simulink model "FOCwithLOAD"  (R2024b)
settings: Solver=FixedStepDiscrete  StartTime=0.0  StopTime=inf  RelTol=1e-3
PreLoadFcn:
  | % 自动加载同目录下的 linear_data.m，确保换机/首次打开可直接更新与编译
  | if ~evalin('base', 'exist(''Ts'',''var'') && exist(''pmsm'',''var'') && exist(''SMRC_I_Vsat_thresh'',''var'')')
  |     mdlDir_ = '';
  |     if bdIsLoaded('FOCwithLOAD'), mdlDir_ = fileparts(get_param('FOCwithLOAD', 'FileName')); end
  |     if isempty(mdlDir_), mdlDir_ = fileparts(which('FOCwithLOAD')); end
  |     if isempty(mdlDir_), mdlDir_ = pwd; end
  |     dataFile_ = fullfile(mdlDir_, 'linear_data.m');
  |     if isfile(dataFile_)
  |         assignin('base', 'linearDataFileTmp_', dataFile_);
  |         evalin('base', 'run(linearDataFileTmp_); clear linearDataFileTmp_');
  |     end
  |     clear mdlDir_ dataFile_
  | end
InitFcn:
  | % 自动加载同目录下的 linear_data.m，确保换机/首次打开可直接更新与编译
  | if ~evalin('base', 'exist(''Ts'',''var'') && exist(''pmsm'',''var'') && exist(''SMRC_I_Vsat_thresh'',''var'')')
  |     mdlDir_ = '';
  |     if bdIsLoaded('FOCwithLOAD'), mdlDir_ = fileparts(get_param('FOCwithLOAD', 'FileName')); end
  |     if isempty(mdlDir_), mdlDir_ = fileparts(which('FOCwithLOAD')); end
  |     if isempty(mdlDir_), mdlDir_ = pwd; end
  |     dataFile_ = fullfile(mdlDir_, 'linear_data.m');
  |     if isfile(dataFile_)
  |         assignin('base', 'linearDataFileTmp_', dataFile_);
  |         evalin('base', 'run(linearDataFileTmp_); clear linearDataFileTmp_');
  |     end
  |     clear mdlDir_ dataFile_
  | end
values from neighbouring files (symbols this model uses):
  a_hat = Kt_eff / (pmsm.J * omega_pu_base)    [linear_data.m]
  ADRC_B0 = 6055    [linear_data.m]
  ADRC_Wc = 3.2e-3    (= 0.0032)    [linear_data.m]
  ADRC_Wo = 30    [linear_data.m]
  alpha_ppc = exp(-lambda_ppc*Ts_speed)    [linear_data.m]
  b_hat = pmsm.B/pmsm.J    [linear_data.m]
  beta1 = single(2.0 * w_o)    [linear_data.m]
  beta2_sat_scale = 0.2    [linear_data.m]
  dataType = 'single'    [linear_data.m]
  gamma_reset = 0.9    [linear_data.m]
  inv_a_hat = 1/double(a_hat)    [linear_data.m]
  k_xi = 55    [linear_data.m]
  Kff = 0.98931745    [linear_data.m]
  lambda_ppc = 45    [linear_data.m]
  P_inf_const = 0.004    [linear_data.m]
  PI_params = mcb_SetControllerParameters(pmsm,inverter,PU_System,T_pwm,Ts,Ts_speed)    [linear_data.m]
  pmsm2 = pmsm    [linear_data.m]
  s_limit_sat = 0.9    [linear_data.m]
  speedRPM2mmps = pmlsm.mmps_per_rpm    [linear_data.m]
  target = mcb_SetProcessorDetails('F28379D',PWM_frequency)    [linear_data.m]
  Ts = T_pwm    (= 5e-05)    [linear_data.m]
  Ts_motor = T_pwm/2    (= 2.5e-05)    [linear_data.m]
  Ts_speed = 1*Ts    (= 5e-05)    [linear_data.m]
  w_o = single(200.0)    [linear_data.m]
  z2_limit = single(100.0)    [linear_data.m]
undefined symbols (not defined in the file or in its folder): DiscIntNeverNeededParam, Down, GPTRIP1SEL, GPTRIP2SEL, innerPI, inverter, inverter2, outerPI, pmlsm, pmsm, Tctr, TZ1, TZ2, Up
libraries: c2802xlib x13, simulink x10, c2837xDlib x6, c280xlib x6, slpidlib x5, svdschedulerlib x4, mcbcontrolslib x4, mcbpositiondecoderlib x2, mcbpmsmnonlinearlib x2, autolibpmsmexterior x2, mcbplantlib x2, svdutilitieslib x1
(part 1 of 5)
settings Model: ExtModeTrigDuration=8  Creator=The MathWorks, Inc.  LastModifiedBy=admin
settings SolverCC: AlgebraicLoopSolver=TrustRegion  MaxZcPerStep=1
settings OptimizationCC: DefaultParameterBehavior=Inlined  DefaultUnderspecifiedDataType=single  ReuseModelBlockBuffer=off  EnhancedBackFolding=on  InitFltsAndDblsToZero=on  NoFixptDivByZeroProtection=on  EfficientFloat2IntCast=on  EfficientMapNaN2IntZero=off  MaxStackSize=1024  OptimizeBlockOrder=speed  DifferentSizesBufferReuse=on  DenormalBehavior=FlushToZero  EfficientTunableParamExpr=on
settings DebuggingCC: MultiTaskDSMMsg=none  ParameterPrecisionLossMsg=none  ParameterTunabilityLossMsg=error  UnconnectedInputMsg=warning  UnconnectedOutputMsg=warning  UnconnectedLineMsg=warning
settings HardwareCC: ProdBitPerChar=16  ProdBitPerInt=16  ProdBitPerPointer=32  ProdBitPerSizeT=32  ProdBitPerPtrDiffT=32  ProdLargestAtomicInteger=Integer  ProdLargestAtomicFloat=None  ProdWordSize=16  ProdLongLongMode=on  ProdHWDeviceType=Texas Instruments->C2000
settings ModelReferenceCC: EnableRefExpFcnMdlSchedulingChecks=on
settings SFSimCC: MATLABDynamicMemAlloc=off
settings RTWCC: Description=Embedded Coder  SystemTargetFile=ert.tlc  HardwareBoard=TI Delfino F28379D LaunchPad  TemplateMakefile=ert_default_tmf  GenerateReport=on  Toolchain=Texas Instruments Code Composer Studio (C2000)  BuildConfiguration=Faster Runs  GPUComputeCapability=3.5  DLArmComputeVersion=19.05
settings CodeAppCC: IgnoreCustomStorageClasses=off  StateflowObjectComments=on
settings ERTTargetCC: CodeReplacementLibrary=TI C28x  ExtModeStaticAllocSize=10000  InlinedParameterPlacement=Hierarchical  ConvertIfToSwitch=off  SuppressUnreachableDefaultCases=off  MemSecPackage=tic2000demospkg  DynamicArrayContainerType=coder::array

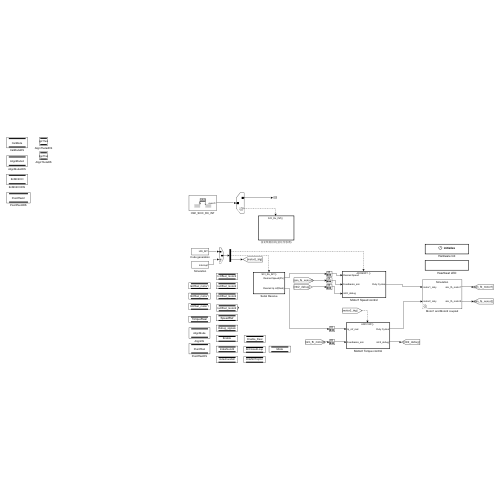
[thumbnail: Simulink's stored preview of the top-level diagram]
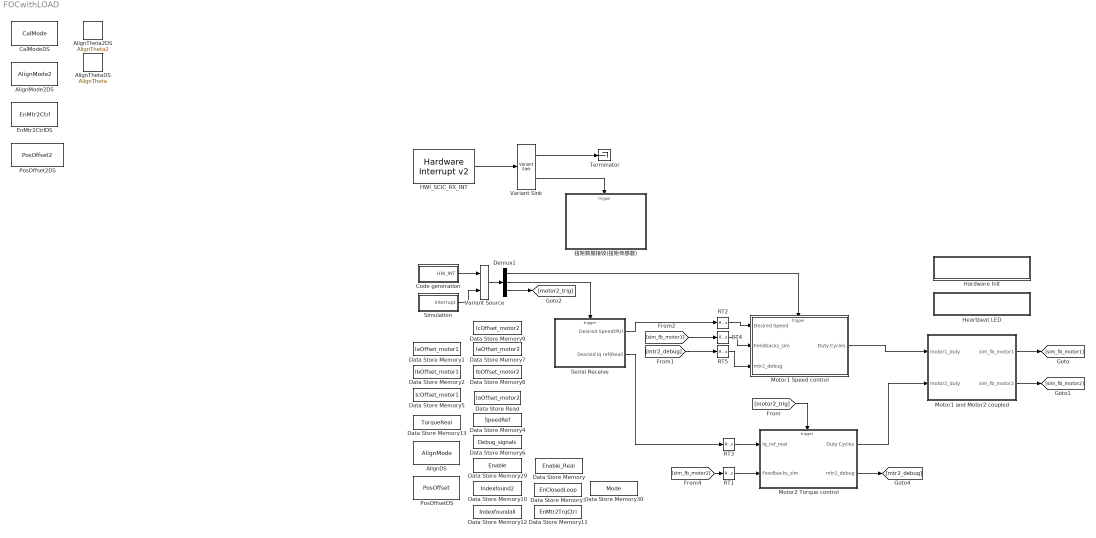
== system FOCwithLOAD ==
  AlignDS : DataStoreMemory  DataStoreName=AlignMode  WriteAfterWriteMsg=warning  ShowAdditionalParam=off  OutDataTypeStr=boolean
  AlignMode2DS : DataStoreMemory  DataStoreName=AlignMode2  WriteAfterWriteMsg=warning  ShowAdditionalParam=off  OutDataTypeStr=boolean
  AlignTheta2DS : DataStoreMemory  DataStoreName=AlignTheta2  WriteAfterWriteMsg=warning  ShowAdditionalParam=off  OutDataTypeStr=single
  AlignThetaDS : DataStoreMemory  DataStoreName=AlignTheta  WriteAfterWriteMsg=warning  ShowAdditionalParam=off  OutDataTypeStr=single
  CalModeDS : DataStoreMemory  DataStoreName=CalMode  WriteAfterWriteMsg=warning  ShowAdditionalParam=off  OutDataTypeStr=uint8
  Code generation : Subsystem
  Data Store Memory : DataStoreMemory  DataStoreName=Enable_Real  WriteAfterWriteMsg=warning  ShowAdditionalParam=off
  Data Store Memory1 : DataStoreMemory  DataStoreName=IaOffset_motor1  ReadBeforeWriteMsg=warning  WriteAfterWriteMsg=warning  WriteAfterReadMsg=warning  InitialValue=inverter.CtSensAOffset  ShowAdditionalParam=off
  Data Store Memory10 : DataStoreMemory  DataStoreName=Indexfound2  ReadBeforeWriteMsg=warning  WriteAfterWriteMsg=warning  WriteAfterReadMsg=warning  ShowAdditionalParam=off  OutDataTypeStr=boolean
  Data Store Memory11 : DataStoreMemory  DataStoreName=EnMtr2TrqCtrl  ReadBeforeWriteMsg=warning  WriteAfterWriteMsg=warning  WriteAfterReadMsg=warning  ShowAdditionalParam=off  OutDataTypeStr=boolean
  Data Store Memory12 : DataStoreMemory  DataStoreName=Indexfoundall  ReadBeforeWriteMsg=warning  WriteAfterWriteMsg=warning  WriteAfterReadMsg=warning  ShowAdditionalParam=off  OutDataTypeStr=boolean
  Data Store Memory13 : DataStoreMemory  DataStoreName=TorqueReal  InitialValue=1  ShowAdditionalParam=off  OutDataTypeStr=single
  Data Store Memory2 : DataStoreMemory  DataStoreName=IbOffset_motor1  ReadBeforeWriteMsg=warning  WriteAfterWriteMsg=warning  WriteAfterReadMsg=warning  InitialValue=inverter.CtSensBOffset  ShowAdditionalParam=off
  Data Store Memory29 : DataStoreMemory  DataStoreName=Enable  ReadBeforeWriteMsg=warning  WriteAfterWriteMsg=warning  WriteAfterReadMsg=warning  ShowAdditionalParam=off  OutDataTypeStr=boolean
  Data Store Memory3 : DataStoreMemory  DataStoreName=EnClosedLoop  ReadBeforeWriteMsg=warning  WriteAfterWriteMsg=warning  WriteAfterReadMsg=warning  ShowAdditionalParam=off  OutDataTypeStr=boolean
  Data Store Memory4 : DataStoreMemory  DataStoreName=SpeedRef  ShowAdditionalParam=off
  Data Store Memory5 : DataStoreMemory  DataStoreName=IcOffset_motor1  ReadBeforeWriteMsg=warning  WriteAfterWriteMsg=warning  WriteAfterReadMsg=warning  InitialValue=inverter.CtSensCOffset  ShowAdditionalParam=off
  Data Store Memory6 : DataStoreMemory  DataStoreName=Debug_signals  ReadBeforeWriteMsg=warning  WriteAfterWriteMsg=warning  WriteAfterReadMsg=warning  InitialValue=5  ShowAdditionalParam=off  OutDataTypeStr=uint16
  Data Store Memory7 : DataStoreMemory  DataStoreName=IaOffset_motor2  ReadBeforeWriteMsg=warning  WriteAfterWriteMsg=warning  WriteAfterReadMsg=warning  InitialValue=inverter2.CtSensAOffset  ShowAdditionalParam=off
  Data Store Memory8 : DataStoreMemory  DataStoreName=IbOffset_motor2  ReadBeforeWriteMsg=warning  WriteAfterWriteMsg=warning  WriteAfterReadMsg=warning  InitialValue=inverter2.CtSensBOffset  ShowAdditionalParam=off
  Data Store Memory9 : DataStoreMemory  DataStoreName=IcOffset_motor2  ReadBeforeWriteMsg=warning  WriteAfterWriteMsg=warning  WriteAfterReadMsg=warning  InitialValue=inverter2.CtSensCOffset  ShowAdditionalParam=off
  Data Store Read : DataStoreRead  DataStoreName=IaOffset_motor2  IndexOptions=Index vector (dialog)  Indices=1  OutputSizes=1
  Data Store Memory30 : DataStoreMemory  DataStoreName=Mode  ReadBeforeWriteMsg=warning  WriteAfterWriteMsg=warning  WriteAfterReadMsg=warning  InitialValue=uint16(0)  ShowAdditionalParam=off  OutDataTypeStr=uint16
  Demux1 : Demux  Outputs=3
  EnMtr2CtrlDS : DataStoreMemory  DataStoreName=EnMtr2Ctrl  WriteAfterWriteMsg=warning  ShowAdditionalParam=off  OutDataTypeStr=boolean
  HWI_SCIC_RX_INT : svdschedulerlib/Hardware Interrupt v2  ISRGroup=ADC - Analog to Digital Converter  ISRName=ADCA1_INT  ISRNumber=32  NumEventsToServe=1  EventsList={'on','EOC event','1';'off','Overflow event','2';'off','Custom event','3'}  SelectedEvents={'event1'}  TaskPriority=20  DisablePreemption=on  ClearInterruptFlagsAtEndOfEvent=on  InterruptDefinitionFile=$(TARGET_ROOT)/registry/interrupts/F2837xS_interrupts.xml  HardwareBoard=F2837x  EnableSimPort=off
      settings: LibrarySourceBlock=c2000lib/Scheduling/Hardware Interrupt
  Hardware Init : Subsystem  TreatAsAtomicUnit=on
  Heartbeat LED : Subsystem  TreatAsAtomicUnit=on
  Motor1 Speed control : Subsystem
      settings: RTWSystemCode=Nonreusable function
  Motor1 and Motor2 coupled : Subsystem  Variant=on  VariantControlMode=sim codegen switching  VariantControl=Motor1 and Motor2 coupled
  Motor2 Torque control : Subsystem
      settings: RTWSystemCode=Nonreusable function
  PosOffset2DS : DataStoreMemory  DataStoreName=PosOffset2  WriteAfterWriteMsg=warning  ShowAdditionalParam=off  OutDataTypeStr=single
  PosOffsetDS : DataStoreMemory  DataStoreName=PosOffset  WriteAfterWriteMsg=warning  ShowAdditionalParam=off  OutDataTypeStr=single
  RT{1..5} (5 alike) : RateTransition  Deterministic=off
  Serial Receive : Subsystem  SystemSampleTime=1e-3
  Simulation : Subsystem
  Terminator : Terminator
  Variant Sink : VariantSink  VariantControlMode=sim codegen switching
  Variant Source : VariantSource  VariantControlMode=sim codegen switching  OutputFunctionCall=on
  扭矩数据接收(扭矩传感器) : Subsystem  SystemSampleTime=1e-3
  wires:
  RT4/1 -> Motor1 Speed control/2(Feedbacks_sim)
  [sim_fb_motor1] -> RT4/1
  Simulation/1(Interrupt) -> Variant Source/2
  Code generation/1(HW_INT) -> Variant Source/1
  Variant Source/1 -> Demux1/1
  Demux1/1 -> Motor1 Speed control/Trigger
  Demux1/2 -> Serial Receive/Trigger
  Demux1/3 -> [motor2_trig]
  [motor2_trig] -> Motor2 Torque control/Trigger
  [sim_fb_motor2] -> RT1/1
  RT1/1 -> Motor2 Torque control/2(Feedbacks_sim)
  Serial Receive/1(Desired Speed(PU)) -> RT2/1
  Serial Receive/2(Desried Iq ref(Real)) -> RT3/1
  RT2/1 -> Motor1 Speed control/1(Desired Speed)
  RT3/1 -> Motor2 Torque control/1(Iq_ref_real)
  Motor2 Torque control/2(mtr2_debug) -> [mtr2_debug]
  [mtr2_debug] -> RT5/1
  RT5/1 -> Motor1 Speed control/3(mtr2_debug)
  HWI_SCIC_RX_INT/1 -> Variant Sink/1
  Variant Sink/2 -> 扭矩数据接收(扭矩传感器)/Trigger
  Variant Sink/1 -> Terminator/1
  Motor1 Speed control/1(Duty Cycles) -> Motor1 and Motor2 coupled/1(motor1_duty)
  Motor2 Torque control/1(Duty Cycles) -> Motor1 and Motor2 coupled/2(motor2_duty)
  Motor1 and Motor2 coupled/1(sim_fb_motor1) -> [sim_fb_motor1]
  Motor1 and Motor2 coupled/2(sim_fb_motor2) -> [sim_fb_motor2]

== system FOCwithLOAD/Code generation ==
  HWI_ADCB1_INT : svdschedulerlib/Hardware Interrupt v2  ISRGroup=ADC - Analog to Digital Converter  ISRName=ADCA1_INT  ISRNumber=32  NumEventsToServe=1  EventsList={'on','EOC event','1';'off','Overflow event','2';'off','Custom event','3'}  SelectedEvents={'event1'}  TaskPriority=30  DisablePreemption=off  ClearInterruptFlagsAtEndOfEvent=on  InterruptDefinitionFile=$(TARGET_ROOT)/registry/interrupts/F2837xS_interrupts.xml  HardwareBoard=F2837x  EnableSimPort=off
      settings: LibrarySourceBlock=c2000lib/Scheduling/Hardware Interrupt
  HWI_ADCC1_INT : svdschedulerlib/Hardware Interrupt v2  ISRGroup=ADC - Analog to Digital Converter  ISRName=ADCA1_INT  ISRNumber=32  NumEventsToServe=1  EventsList={'on','EOC event','1';'off','Overflow event','2';'off','Custom event','3'}  SelectedEvents={'event1'}  TaskPriority=35  DisablePreemption=off  ClearInterruptFlagsAtEndOfEvent=on  InterruptDefinitionFile=$(TARGET_ROOT)/registry/interrupts/F2837xS_interrupts.xml  HardwareBoard=F2837x  EnableSimPort=off
      settings: LibrarySourceBlock=c2000lib/Scheduling/Hardware Interrupt
  HWI_SCIA_RX_INT : svdschedulerlib/Hardware Interrupt v2  ISRGroup=ADC - Analog to Digital Converter  ISRName=ADCA1_INT  ISRNumber=32  NumEventsToServe=1  EventsList={'on','EOC event','1';'off','Overflow event','2';'off','Custom event','3'}  SelectedEvents={'event1'}  TaskPriority=50  DisablePreemption=off  ClearInterruptFlagsAtEndOfEvent=on  InterruptDefinitionFile=$(TARGET_ROOT)/registry/interrupts/F2837xS_interrupts.xml  HardwareBoard=F2837x  EnableSimPort=off
      settings: LibrarySourceBlock=c2000lib/Scheduling/Hardware Interrupt
  Mux : Mux  Inputs=3
  HW_INT : Outport
  wires:
  HWI_ADCB1_INT/1 -> Mux/1
  HWI_SCIA_RX_INT/1 -> Mux/2
  HWI_ADCC1_INT/1 -> Mux/3
  Mux/1 -> HW_INT/1

== system FOCwithLOAD/Hardware Init ==
  Event Listener : EventListener  DisableCoverage=on  EventName=reset
  Variant Subsystem : Subsystem  Variant=on  VariantControlMode=sim codegen switching

== system FOCwithLOAD/Heartbeat LED ==
  note: Heartbeat LED 1HZ
  Heartbeat LED : Subsystem  Variant=on  VariantControlMode=sim codegen switching
  RED_LED : Constant  OutDataTypeStr=uint16  SampleTime=0.5
  wires:
  RED_LED/1 -> Heartbeat LED/1(In1)

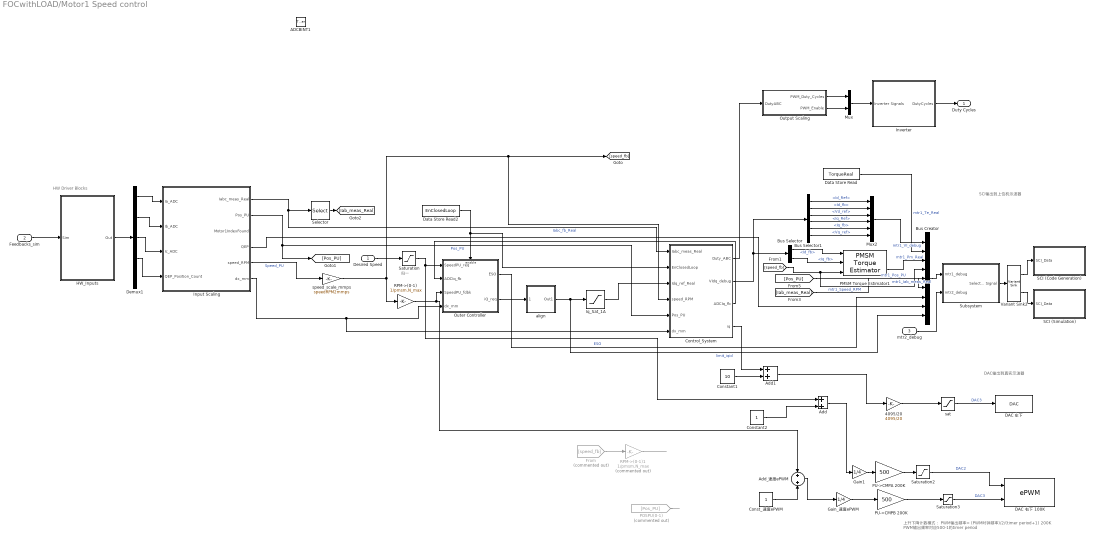
== system FOCwithLOAD/Motor1 Speed control ==
  note: 归一
  note: DAC输出到真实示波器
  note: HW Driver Blocks
  note: SCI输出到上位机示波器
  note: 上升下降计数模式： PWM输出频率= (PWM时钟频率)/2/(timer period+1)
      | 200K PWM输出频率对应500-1的timer period
  Desired Speed : Inport
  Feedbacks_sim : Inport  Port=2
  mtr2_debug : Inport  Port=3
  "ADCBINT1 " : TriggerPort  TriggerType=function-call  VariantControl=Variant  PortDimensions=1
  4095/20 : Gain  Gain=4095/20
  Add : Sum
  Add1 : Sum
  Add_速度ePWM : Sum
  Bus Creator : BusCreator  Inputs=9
  Bus Selector : BusSelector  OutputSignals=Id_fb,Iq_fb
  Bus Selector1 : BusSelector  OutputSignals=Id_Ref,Id_fb,Vd_ref,Iq_Ref,Iq_fb,Vq_ref
  Const_速度ePWM : Constant
  Constant1 : Constant  Value=10  OutDataTypeStr=single
  Constant2 : Constant  OutDataTypeStr=single
  Control_System : Subsystem
  DAC 右下 100K : c2802xlib/ePWM  PwmType=C2000_Type4  useModule=ePWM7  ePWMxLINKTBPRD=Not Linked  periodUnits=Clock cycles  timerSource=Specify via dialog  timerPeriod_clk=300-1  timerPeriod_sec=0.0001  tbshadow=Counter equals to zero  countingMode=Up-Down  phaseActiveEnable=Disable  phaseDirection=Count down after sync  phaseActive=0  synchronizationEnable=off  dcaevt1Sync=off  dcbevt1Sync=off  synchronizationOption=Disable  dcbevt1SyncOut=off  dcaevt1SyncOut=off  cmpdSyncOut=off  cmpcSyncOut=off  cmpbSyncOut=off  zeroSyncOut=off  swfSyncOut=off  perSynchronizationOption=Counter equals to period (CTR=PRD)  clockPrescale=1  HSclockPrescale=1  enswap=off  ePWMxAStatus=on  ePWMxAactionLogic1=Set  ePWMxAactionLogic2=Clear  ePWMxAactionLogic3=Clear  ePWMxAactionLogic4=Set  ePWMxAactionLogic5=Do nothing  ePWMxAactionLogic6=Do nothing  ePWMxACSFenable=off  ePWMxACSFvalue=Forcing disable  ePWMxASFreload=Zero  ePWMxBStatus=on  ePWMxBactionLogic1=Set  ePWMxBactionLogic2=Clear  ePWMxBactionLogic3=Do nothing  ePWMxBactionLogic4=Do nothing  ePWMxBactionLogic5=Clear  ePWMxBactionLogic6=Set  ePWMxBCSFenable=off  ePWMxBCSFvalue=Forcing disable  ePWMxBSFreload=Zero  ePWNxBOutWay=off  ePWMxLINKCMPA=Not Linked  CMPAUnits=Clock cycles  CMPASource=Input port  CMPAValue_per=50  CMPAValue_clk=0  enCMPAshadow=Counter equals to zero (CTR=Zero)  ePWMxLINKCMPB=Not Linked  CMPBUnits=Clock cycles  CMPBSource=Input port  CMPBValue_per=50  CMPBValue_clk=0  enCMPBshadow=Counter equals to zero (CTR=Zero)  ePWMxLINKCMPC=Not Linked  CMPCUnits=Clock cycles  CMPCSource=Specify via dialog  CMPCValue_per=50  CMPCValue_clk=32000  enCMPCshadow=Counter equals to zero (CTR=Zero)  ePWMxLINKCMPD=Not Linked  CMPDUnits=Clock cycles  CMPDSource=Specify via dialog  CMPDValue_per=50  CMPDValue_clk=32000  enCMPDshadow=Counter equals to zero (CTR=Zero)  enableDBePWMxA=off  enableDBePWMxB=off  enhalfcycle=off  DBpolarity=Active high (AH)  DBedgeDelay=Positive  DBSource_ePWMxA=ePWMxA  DBSource_ePWMxB=ePWMxA  DBPeriodUnits=Clock cycles  DBperiodSource=Specify via dialog  REDperiod=0  FEDperiod=0  REDperiod_sec=0  FEDperiod_sec=0  LoadModeDBRED=Immediate without using shadow  LoadModeDBFED=Immediate without using shadow  adcstartModuleA=off  adcrequestEventA=First event  adcstartEventA=Digital Compare Module A Event 1 start of conversion (DCAEVT1.soc)  adcstartEventA_type2=Counter equals to zero (CTR=Zero)  adcstartModuleB=off  adcrequestEventB=First event  adcstartEventB=Counter equals to zero (CTR=Zero)  adcstartEventB_type2=Counter equals to zero (CTR=Zero)  intEn=off  intPrd=First event  intSel=Counter equals to zero (CTR=Zero)  intSel_type2=Counter equals to zero (CTR=Zero)  hrpe=off  enHRPWM=off  HRPWM_LoadMode=Counter equals to period (CTR=PRD)  HRPWM_CTLMode=Duty or Period control mode  HRPWM_EDGMode=Both edge  hrpeb=off  enHRPWMB=off  HRPWM_LoadModeB=Counter equals to zero (CTR=ZERO)  HRPWM_CTLModeB=Duty or Period control mode  HRPWM_EDGModeB=Both edge  enHRDBRED=off  enHRDBFED=off  enSFO=on  enautoconv=on  chopperEnable=off  chopperFrequency=1  chopperFirstwidth=1  chopperDuty=12.5%  tripZonesource=Specify via dialog  tzselOSHT1=off  tzselOSHT2=off  tzselOSHT3=off  tzselOSHT4=off  tzselOSHT5=off  tzselOSHT6=off  tzselOSHDCAEV1=off  tzselOSHDCBEV1=off  tzselCBC1=off  tzselCBC2=off  tzselCBC3=off  tzselCBC4=off  tzselCBC5=off  tzselCBC6=off  tzselCBCDCAEV2=off  tzselCBCDCBEV2=off  enTzOstIntr=off  enTzCbcIntr=off  enTzDCAEVT1Intr=off  enTzDCAEVT2Intr=off  enTzDCBEVT1Intr=off  enTzDCBEVT2Intr=off  tzclrCBCLatch=Counter equals to zero (CTR=Zero)  ePWMxAforced=No action  ePWMxBforced=No action  DCAEVT1forced=No action  DCBEVT1forced=No action  DCAEVT2forced=No action  DCBEVT2forced=No action  dcah=Trip Zone 1 input (TZ1)  dcal=Trip Zone 2 input (TZ2)  dcbh=Trip Zone 1 input (TZ1)  dcbl=Trip Zone 2 input (TZ2)  dcah_type2=GPTRIP1SEL/(TZ1)  dcal_type2=GPTRIP1SEL/(TZ1)  dcbh_type2=GPTRIP1SEL/(TZ1)  dcbl_type2=GPTRIP1SEL/(TZ1)  gendcaevt1=Event disabled  gendcaevt2=Event disabled  gendcbevt1=Event disabled  gendcbevt2=Event disabled  dcaevt1src=DCAEVT1 with sync  dcaevt2src=DCAEVT2 with sync  dcbevt1src=DCBEVT1 with sync  dcbevt2src=DCBEVT2 with sync  pulsesel=Counter equals to zero (CTR=Zero)  blankinv=off  blankoffset=0  blankwidth=0  evsrcsel=Filtered version of DCAEVT1 (DCAEVT1FILT)  encape=off
      settings: LibrarySourceBlock=c2837xDlib/ePWM
  DAC 左下 : c2837xDlib/DAC  channel=B  saturate=on
  Data Store Read : DataStoreRead  DataStoreName=TorqueReal  IndexOptions=Index vector (dialog)  Indices=1  OutputSizes=1
  Data Store Read2 : DataStoreRead  DataStoreName=EnClosedLoop  IndexOptions=Index vector (dialog)  Indices=1  OutputSizes=1
  Demux1 : Demux  Outputs=5
  From : From  Commented=on  GotoTag=speed_fb
  Gain1 : Gain  Gain=1/4
  Gain_速度ePWM : Gain  Gain=1/4
  HW_Inputs : Subsystem  Variant=on  VariantControlMode=sim codegen switching
  Input Scaling : Subsystem
  Inverter : Subsystem  Variant=on  VariantControlMode=sim codegen switching
  Iq_Sat_1A : Saturate  UpperLimit=3  LowerLimit=-3
  Mux : Mux  Inputs=2
  Mux2 : Mux  Inputs=6
  Outer Controller : Subsystem
  Output Scaling : Subsystem
  PMSM Torque Estimator1 : mcbpmsmnonlinearlib/PMSM Torque Estimator  polePairs=pmsm.p  nonLinearityChoice=Linear model with lumped parameters  Ld=pmsm.Ld  Lq=pmsm.Lq  FluxPM=pmsm.FluxPM  idVec=[-40, -20, 0, 20]  iqVec=[-40, -20, 0, 20, 40]  LdTable=0.2e-3 * ones(4, 5)  LqTable=0.2e-3 * ones(4, 5)  FluxPMTable=6.4e-3 * ones(4, 5)  FluxDTable=[-1.6,-1.6,-1.6,-1.6,-1.6;2.4,2.4,2.4,2.4,2.4;6.4,6.4,6.4,6.4,6.4;10.4,10.4,10.4,10.4,10.4]*1e-3  FluxQTable=[-8,-4,0,4,8;-8,-4,0,4,8;-8,-4,0,4,8;-8,-4,0,4,8]*1e-3  Units=SI Units  V_base=PU_System_motor1.V_base  I_base=PU_System_motor1.I_base  N_base=PU_System_motor1.N_base  T_base=1  P_base=1  scaledTables=on
  POSPU(0-1) : From  Commented=on  GotoTag=Pos_PU
  PU->CMPA 200K : Gain  Gain=500
  PU->CMPB 200K : Gain  Gain=500
  RPM->(0-1) : Gain  Gain=1/pmsm.N_max
  RPM->(0-1)1 : Gain  Commented=on  Gain=1/pmsm.N_max
  SCI (Code Generation) : Subsystem
  SCI (Simulation) : Subsystem
  Saturation : Saturate  UpperLimit=1  LowerLimit=-1
  Saturation2 : Saturate  UpperLimit=500  LowerLimit=0
  Saturation3 : Saturate  UpperLimit=500  LowerLimit=0
  Selector : Selector  InputPortWidth=3  IndexOptions=Index vector (dialog)  Indices=[1 2]  OutputSizes=1
  Subsystem : Subsystem
  Variant Sink2 : VariantSink  VariantControlMode=sim codegen switching
  align : Subsystem
  sat : Saturate  UpperLimit=4095  LowerLimit=0
  speed_scale_mmps : Gain  Gain=speedRPM2mmps
  Duty Cycles : Outport  InitialOutput=0  VectorParamsAs1DForOutWhenUnconnected=off
  wires:
  HW_Inputs/1(Out) -> Demux1/1
  Feedbacks_sim/1 -> HW_Inputs/1(Sim)
  Desired Speed/1 -> Saturation/1
  RPM->(0-1)/1 -> Outer Controller/3(SpeedPU_fdbk), Add_速度ePWM/1
  Saturation/1 -> Add/1, Outer Controller/1(SpeedPU_req)
  Saturation3/1 -> DAC 右下 100K/2  "DAC3"
  Saturation2/1 -> DAC 右下 100K/1  "DAC2"
  PU->CMPA 200K/1 -> Saturation2/1
  PU->CMPB 200K/1 -> Saturation3/1
  POSPU(0-1)/1 -> ?
  From/1 -> RPM->(0-1)1/1
  Add/1 -> Gain1/1
  RPM->(0-1)1/1 -> ?
  Constant2/1 -> Add/2
  4095/20/1 -> sat/1
  sat/1 -> DAC 左下/1  "DAC3"
  Gain1/1 -> PU->CMPA 200K/1
  Selector/1 -> [Iab_meas_Real]
  Demux1/3 -> Input Scaling/3(Ic_ADC)
  Demux1/1 -> Input Scaling/1(Ia_ADC)
  Demux1/2 -> Input Scaling/2(Ib_ADC)
  Input Scaling/5(speed_RPM) -> speed_scale_mmps/1  "Speed_PU"
  Demux1/4 -> Input Scaling/4(QEP_Position_Count)
  align/1(Out1) -> Bus Creator/9, Iq_Sat_1A/1  "limit_iqid"
  Output Scaling/1(PWM_Duty_Cycles) -> Mux/1
  Mux/1 -> Inverter/1(Inverter Signals)
  Inverter/1(DutyCycles) -> Duty Cycles/1
  Input Scaling/1(Iabc_meas_Real) -> Control_System/1(Iabc_meas_Real), Selector/1  "Iabc_fb_Real"
  Input Scaling/2(Pos_PU) -> [Pos_PU], Control_System/5(Pos_PU)  "Pos_PU"
  Control_System/1(Duty_ABC) -> Output Scaling/1(DutyABC)
  Output Scaling/2(PWM_Enable) -> Mux/2
  Data Store Read2/1 -> Outer Controller/Enable, Control_System/2(EnClosedLoop)
  Control_System/2(VIdq_debug) -> Bus Selector/1, Bus Selector1/1
  Control_System/3(ADCIq_fb) -> Outer Controller/2(ADCIq_fb)
  speed_scale_mmps/1 -> Control_System/4(speed_RPM), [speed_fb], RPM->(0-1)/1
  Outer Controller/1(ESO) -> Bus Creator/7  "ESO"
  Data Store Read/1 -> Bus Creator/2  "mtr1_Te_Real"
  [Pos_PU] -> Bus Creator/6  "mtr1_Pos_PU"
  Bus Selector1/1 -> Mux2/1  "<Id_Ref>"
  Variant Sink2/1 -> SCI (Code Generation)/1(SCI_Data)
  Bus Selector1/3 -> Mux2/3  "<Vd_ref>"
  Mux2/1 -> Bus Creator/1  "mtr1_VI_debug"
  Bus Selector1/4 -> Mux2/4  "<Iq_Ref>"
  Bus Creator/1 -> Subsystem/1(mtr1_debug)
  Bus Selector1/6 -> Mux2/6  "<Vq_ref>"
  PMSM Torque Estimator1/2 -> Bus Creator/3  "mtr1_Pm_Real"
  Bus Selector/2 -> PMSM Torque Estimator1/2  "<Iq_fb>"
  Bus Selector/1 -> PMSM Torque Estimator1/1  "<Id_fb>"
  mtr2_debug/1 -> Subsystem/2(mtr2_debug)
  Variant Sink2/2 -> SCI (Simulation)/1(SCI_Data)
  Subsystem/1(Selected Signal) -> Variant Sink2/1
  Bus Selector1/2 -> Mux2/2  "<Id_fb>"
  [speed_fb] -> Bus Creator/4, PMSM Torque Estimator1/3  "mtr1_Speed_RPM"
  [Iab_meas_Real] -> Bus Creator/5  "mtr1_Iab_meas_Real"
  Bus Selector1/5 -> Mux2/5  "<Iq_fb>"
  Iq_Sat_1A/1 -> Control_System/3(Idq_ref_Real)
  Outer Controller/2(iQ_req) -> align/1(real_Iq_input)
  Const_速度ePWM/1 -> Add_速度ePWM/2
  Add_速度ePWM/1 -> Gain_速度ePWM/1
  Gain_速度ePWM/1 -> PU->CMPB 200K/1
  Input Scaling/6(dx_mm) -> Control_System/6(dx_mm), Outer Controller/4(dx_mm)
  Input Scaling/4(QEP) -> Bus Creator/8
  Add1/1 -> 4095/20/1
  Constant1/1 -> Add1/2
  Control_System/4(iq) -> Add1/1

== system FOCwithLOAD/Motor1 and Motor2 coupled ==
  motor1_duty : Inport
  motor2_duty : Inport  Port=2
  Code Generation : Subsystem  VariantControl=(codegen)
  Simulation : Subsystem  VariantControl=(sim)
  sim_fb_motor1 : Outport
  sim_fb_motor2 : Outport  Port=2

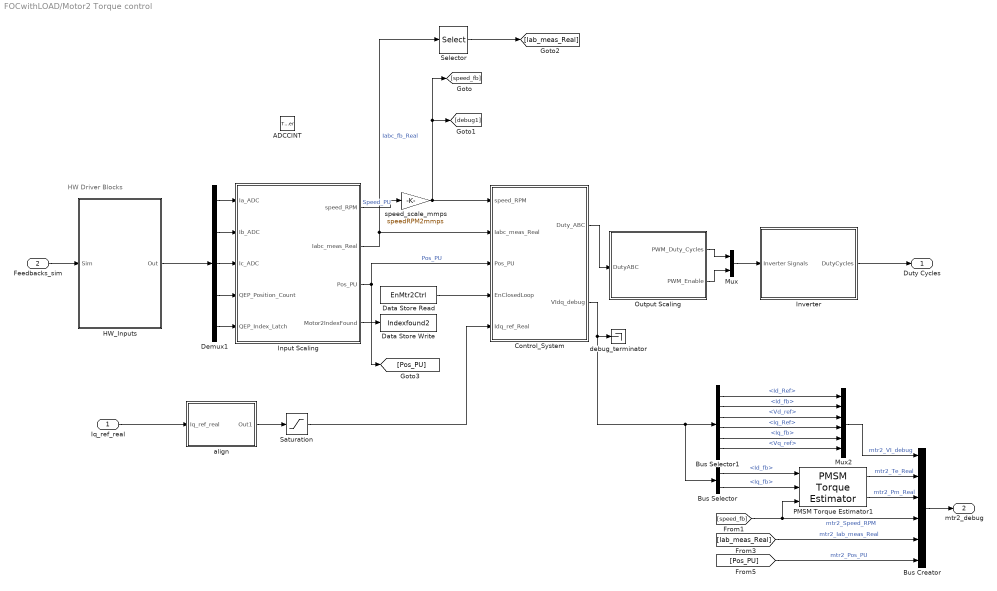
== system FOCwithLOAD/Motor2 Torque control ==
  note: HW Driver Blocks
  Iq_ref_real : Inport
  Feedbacks_sim : Inport  Port=2
  ADCCINT : TriggerPort  TriggerType=function-call  VariantControl=Variant  PortDimensions=1
  Bus Creator : BusCreator  Inputs=6
  Bus Selector : BusSelector  OutputSignals=Id_fb,Iq_fb
  Bus Selector1 : BusSelector  OutputSignals=Id_Ref,Id_fb,Vd_ref,Iq_Ref,Iq_fb,Vq_ref
  Control_System : Subsystem
  Data Store Read : DataStoreRead  DataStoreName=EnMtr2Ctrl  IndexOptions=Index vector (dialog)  Indices=1  OutputSizes=1
  Data Store Write : DataStoreWrite  DataStoreName=Indexfound2  IndexOptions=Index vector (dialog)  Indices=1  OutputSizes=1
  Demux1 : Demux  Outputs=5
  HW_Inputs : Subsystem  Variant=on  VariantControlMode=sim codegen switching
  Input Scaling : Subsystem
  Inverter : Subsystem  Variant=on  VariantControlMode=sim codegen switching
  Mux : Mux  Inputs=2
  Mux2 : Mux  Inputs=6
  Output Scaling : Subsystem
  PMSM Torque Estimator1 : mcbpmsmnonlinearlib/PMSM Torque Estimator  polePairs=pmsm.p  nonLinearityChoice=Linear model with lumped parameters  Ld=pmsm.Ld  Lq=pmsm.Lq  FluxPM=pmsm.FluxPM  idVec=[-40, -20, 0, 20]  iqVec=[-40, -20, 0, 20, 40]  LdTable=0.2e-3 * ones(4, 5)  LqTable=0.2e-3 * ones(4, 5)  FluxPMTable=6.4e-3 * ones(4, 5)  FluxDTable=[-1.6,-1.6,-1.6,-1.6,-1.6;2.4,2.4,2.4,2.4,2.4;6.4,6.4,6.4,6.4,6.4;10.4,10.4,10.4,10.4,10.4]*1e-3  FluxQTable=[-8,-4,0,4,8;-8,-4,0,4,8;-8,-4,0,4,8;-8,-4,0,4,8]*1e-3  Units=SI Units  V_base=PU_System_motor1.V_base  I_base=PU_System_motor1.I_base  N_base=PU_System_motor1.N_base  T_base=1  P_base=1  scaledTables=on
  Saturation : Saturate  UpperLimit=2.5  LowerLimit=-2.5
  Selector : Selector  InputPortWidth=3  IndexOptions=Index vector (dialog)  Indices=[1 2]  OutputSizes=1
  align : Subsystem
  debug_terminator : Terminator
  speed_scale_mmps : Gain  Gain=speedRPM2mmps
  Duty Cycles : Outport  InitialOutput=0  VectorParamsAs1DForOutWhenUnconnected=off
  mtr2_debug : Outport  Port=2
  wires:
  Control_System/1(Duty_ABC) -> Output Scaling/1(DutyABC)
  Input Scaling/3(Pos_PU) -> [Pos_PU], Control_System/3(Pos_PU)  "Pos_PU"
  Input Scaling/2(Iabc_meas_Real) -> Selector/1, Control_System/2(Iabc_meas_Real)  "Iabc_fb_Real"
  Demux1/1 -> Input Scaling/1(Ia_ADC)
  Demux1/2 -> Input Scaling/2(Ib_ADC)
  Output Scaling/1(PWM_Duty_Cycles) -> Mux/1
  Output Scaling/2(PWM_Enable) -> Mux/2
  Inverter/1(DutyCycles) -> Duty Cycles/1
  HW_Inputs/1(Out) -> Demux1/1
  Feedbacks_sim/1 -> HW_Inputs/1(Sim)
  Demux1/3 -> Input Scaling/3(Ic_ADC)
  Input Scaling/4(Motor2IndexFound) -> Data Store Write/1
  Data Store Read/1 -> Control_System/4(EnClosedLoop)
  Bus Selector1/3 -> Mux2/3  "<Vd_ref>"
  Bus Creator/1 -> mtr2_debug/1
  Bus Selector1/6 -> Mux2/6  "<Vq_ref>"
  Bus Selector/1 -> PMSM Torque Estimator1/1  "<Id_fb>"
  Mux2/1 -> Bus Creator/1  "mtr2_VI_debug"
  PMSM Torque Estimator1/2 -> Bus Creator/3  "mtr2_Pm_Real"
  Bus Selector1/4 -> Mux2/4  "<Iq_Ref>"
  Bus Selector1/2 -> Mux2/2  "<Id_fb>"
  [Pos_PU] -> Bus Creator/6  "mtr2_Pos_PU"
  [speed_fb] -> PMSM Torque Estimator1/3, Bus Creator/4  "mtr2_Speed_RPM"
  Bus Selector1/5 -> Mux2/5  "<Iq_fb>"
  PMSM Torque Estimator1/1 -> Bus Creator/2  "mtr2_Te_Real"
  [Iab_meas_Real] -> Bus Creator/5  "mtr2_Iab_meas_Real"
  Bus Selector1/1 -> Mux2/1  "<Id_Ref>"
  Control_System/2(VIdq_debug) -> Bus Selector/1, Bus Selector1/1, debug_terminator/1
  Bus Selector/2 -> PMSM Torque Estimator1/2  "<Iq_fb>"
  Selector/1 -> [Iab_meas_Real]
  Input Scaling/1(speed_RPM) -> speed_scale_mmps/1  "Speed_PU"
  speed_scale_mmps/1 -> [speed_fb], [debug1], Control_System/1(speed_RPM)
  Demux1/4 -> Input Scaling/4(QEP_Position_Count)
  Demux1/5 -> Input Scaling/5(QEP_Index_Latch)
  Iq_ref_real/1 -> align/1(Iq_ref_real)
  align/1(Out1) -> Saturation/1
  Mux/1 -> Inverter/1(Inverter Signals)
  Saturation/1 -> Control_System/5(Idq_ref_Real)

== system FOCwithLOAD/Serial Receive ==
  note: Simulation Input
  SCI_Rx_INT : TriggerPort  TriggerType=function-call  VariantControl=Variant
  Add1 : Sum  Inputs=++++
  Constant : Constant  Value=300  OutDataTypeStr=single
  Iq_Ref(A) : Step  Time=2  After=0.7  OutDataTypeStr=single
  Parse SCI Rx : Subsystem
  Serial Receive : Subsystem  SystemSampleTime=1e-3
  Signal Packing : Subsystem
  Speed_Ref_CW (rpm) : Step  Time=0  After=1200  OutDataTypeStr=single
  Step1 : Step  Commented=on  Time=0.2  After=0.1  OutDataTypeStr=single
  Step2 : Step  Commented=on  Time=.5  After=-0.1  OutDataTypeStr=single
  Step3 : Step  Commented=on  After=0.3  OutDataTypeStr=single
  Step4 : Step  Commented=on  Time=2  After=-0.3  OutDataTypeStr=single
  Variant Source1 : VariantSource  VariantControlMode=sim codegen switching
  Desired Speed(PU) : Outport
  Desried Iq ref(Real) : Outport  Port=2
  wires:
  Signal Packing/1(Data) -> Variant Source1/2  "Sim"
  Serial Receive/1(Rx) -> Variant Source1/1  "codegen"
  Variant Source1/1 -> Parse SCI Rx/1(Rx)
  Parse SCI Rx/2(Desried Iq ref) -> Desried Iq ref(Real)/1
  Parse SCI Rx/1(Desired Speed) -> Desired Speed(PU)/1
  Add1/1 -> Signal Packing/2(IqRef)
  Step1/1 -> Add1/1
  Step3/1 -> Add1/2
  Step2/1 -> Add1/3
  Step4/1 -> Add1/4
  Constant/1 -> Signal Packing/1(Speedref)

== system FOCwithLOAD/Simulation ==
  Mux : Mux  Inputs=3
  Pulse Generator1 : DiscretePulseGenerator  PulseType=Time based  Period=Ts  PulseWidth=20  PhaseDelay=Ts
  Pulse Generator2 : DiscretePulseGenerator  PulseType=Time based  Period=Ts  PulseWidth=20
  SCI_Rx_INT : simulink/Ports & Subsystems/Function-Call Generator  sample_time=0.001  numberOfIterations=1  DisallowWideOutput=off
  Simulation1 : Subsystem
  Simulation2 : Subsystem
  Interrupt : Outport
  wires:
  Pulse Generator1/1 -> Simulation1/Trigger
  Mux/1 -> Interrupt/1
  SCI_Rx_INT/1 -> Mux/2
  Pulse Generator2/1 -> Simulation2/Trigger
  Simulation2/1(Interrupt) -> Mux/1
  Simulation1/1(Interrupt) -> Mux/3

== system FOCwithLOAD/扭矩数据接收(扭矩传感器) ==
  SCI_Rx_INT : TriggerPort  TriggerType=function-call  VariantControl=Variant
  ASCII to String : ASCIIToString
  Data Store Write : DataStoreWrite  DataStoreName=TorqueReal  IndexOptions=Index vector (dialog)  Indices=1  OutputSizes=1
  SCI Receive : c280xlib/SCI Receive  sciModule=C  dataHead=''  headerCheckMaxCount=16  dataTail=13  dataType=uint8  dataLenOptions=Length via dialog  dataDim=7  maxDataLength=1  initValue=0  errOption=Output the last received value  errValue=0  sampleTime=-1  blockingMode=on  timeOut=0.00875  outputStatus=off
  String to Single : ScanString  Format="\"%f\""
  wires:
  SCI Receive/1 -> ASCII to String/1
  ASCII to String/1 -> String to Single/1
  String to Single/1 -> Data Store Write/1

== system FOCwithLOAD/Hardware Init/Variant Subsystem ==
  Code Generation : Subsystem  VariantControl=(codegen)
  Simulation : Subsystem  VariantControl=(sim)

== system FOCwithLOAD/Heartbeat LED/Heartbeat LED ==
  In1 : Inport
  Code generation : Subsystem  VariantControl=(codegen)
  Simulation : Subsystem  VariantControl=(sim)

== system FOCwithLOAD/Motor1 Speed control/Control_System ==
  Iabc_meas_Real : Inport
  EnClosedLoop : Inport  Port=2
  Idq_ref_Real : Inport  Port=3
  speed_RPM : Inport  Port=4
  Pos_PU : Inport  Port=5
  dx_mm : Inport  Port=6
  AlignReadCS : DataStoreRead  DataStoreName=AlignMode  IndexOptions=Index vector (dialog)  Indices=1  OutputSizes=1
  AlignThetaRead : DataStoreRead  DataStoreName=AlignTheta  IndexOptions=Index vector (dialog)  Indices=1  OutputSizes=1
  And_EnSMRC_I : Logic  AllPortsSameDT=off  OutDataTypeStr=boolean
  Closed Loop Control1 : Subsystem  TreatAsAtomicUnit=on
  Not_Align : Logic  Operator=NOT  Inputs=1  AllPortsSameDT=off  OutDataTypeStr=boolean
  OrEn : Logic  Operator=OR  AllPortsSameDT=off  OutDataTypeStr=boolean
  Switch : Switch  Criteria=u2 > Threshold  Threshold=0.5  SaturateOnIntegerOverflow=off  InputSameDT=off
  ThetaSw : Switch  Criteria=u2 > Threshold  Threshold=0.5  SaturateOnIntegerOverflow=off  InputSameDT=off
  ZeroOL : Constant  Value=0  OutDataTypeStr=single
  Duty_ABC : Outport  VectorParamsAs1DForOutWhenUnconnected=off
  VIdq_debug : Outport  Port=2  VectorParamsAs1DForOutWhenUnconnected=off
  ADCIq_fb : Outport  Port=3
  iq : Outport  Port=4
  wires:
  Iabc_meas_Real/1 -> Closed Loop Control1/1(Iabc)
  Idq_ref_Real/1 -> Closed Loop Control1/4(IdqRef)
  speed_RPM/1 -> Closed Loop Control1/3(Speed(RPM))
  Closed Loop Control1/2(VIdq_debug) -> VIdq_debug/1
  Closed Loop Control1/3(ADRCIq_fb) -> ADCIq_fb/1
  ThetaSw/1 -> Closed Loop Control1/2(Thetae_Sensor(0-1))
  Pos_PU/1 -> ThetaSw/3
  OrEn/1 -> Switch/2, Closed Loop Control1/Enable
  Closed Loop Control1/1(Duty) -> Switch/1
  EnClosedLoop/1 -> OrEn/1, And_EnSMRC_I/1
  Switch/1 -> Duty_ABC/1
  ZeroOL/1 -> Switch/3
  And_EnSMRC_I/1 -> Closed Loop Control1/6(EnSMRC_I)
  Not_Align/1 -> And_EnSMRC_I/2
  dx_mm/1 -> Closed Loop Control1/5(dx_mm)
  AlignReadCS/1 -> Not_Align/1, ThetaSw/2, OrEn/2
  Closed Loop Control1/4(iq) -> iq/1
  AlignThetaRead/1 -> ThetaSw/1

== system FOCwithLOAD/Motor1 Speed control/HW_Inputs ==
  Sim : Inport
  Sensor Driver Blocks (codegen) : Subsystem  VariantControl=(codegen)
  Sensor Driver Blocks (sim) : Subsystem  VariantControl=(sim)
  Out : Outport

== system FOCwithLOAD/Motor1 Speed control/Input Scaling ==
  note: Current Measurements
  note: Position & Speed Measurements
  note: QEP
  Ia_ADC : Inport
  Ib_ADC : Inport  Port=2
  Ic_ADC : Inport  Port=3
  QEP_Position_Count : Inport  Port=4
  " Calculate Position and Speed" : Subsystem
  Calculate Phase Currents : Subsystem
  Iabc_meas_Real : Outport
  Pos_PU : Outport  Port=2
  Motor1IndexFound : Outport  Port=3
  QEP : Outport  Port=4
  speed_RPM : Outport  Port=5
  dx_mm : Outport  Port=6
  wires:
  " Calculate Position and Speed"/2(speed) -> speed_RPM/1
  Calculate Phase Currents/1(Iabc_meas_Real) -> Iabc_meas_Real/1  "Iabc_fb_Real"
  " Calculate Position and Speed"/1(Theta_e) -> Pos_PU/1
  Ia_ADC/1 -> Calculate Phase Currents/1(Ia_ADC)
  Ib_ADC/1 -> Calculate Phase Currents/2(Ib_ADC)
  Ic_ADC/1 -> Calculate Phase Currents/3(Ic_ADC)
  QEP_Position_Count/1 -> " Calculate Position and Speed"/1(QEP_Position_Count)
  " Calculate Position and Speed"/4(theta_pu) -> QEP/1
  " Calculate Position and Speed"/5(dx_mm) -> dx_mm/1

== system FOCwithLOAD/Motor1 Speed control/Inverter ==
  Inverter Signals : Inport
  Code Generation : Subsystem  VariantControl=(codegen)
  Simulation : Subsystem  VariantControl=(sim)
  DutyCycles : Outport  VectorParamsAs1DForOutWhenUnconnected=off

== system FOCwithLOAD/Motor1 Speed control/Outer Controller ==
  note: ADRC
  note: PI
  SpeedPU_req : Inport
  ADCIq_fb : Inport  Port=2
  SpeedPU_fdbk : Inport  Port=3
  dx_mm : Inport  Port=4
  Enable : EnablePort  StatesWhenEnabling=reset
  ESO+PPC : MATLAB Function  Commented=on  TreatAsAtomicUnit=on
  MATLAB Function : MATLAB Function  Commented=on  TreatAsAtomicUnit=on
  Manual Switch : ManualSwitch  Commented=on
  Mux : Mux  Commented=on  Inputs=5
  Scope : Scope  Commented=on
  Scope1 : Scope  Commented=on
  Subsystem : Subsystem
  Subsystem1 : Subsystem  Commented=on
  To Workspace : ToWorkspace  Commented=on  VariableName=data_fixed  SaveFormat=Timeseries  SampleTime=-1
  ppc : Subsystem  Commented=on
  ESO : Outport
  iQ_req : Outport  Port=2
  wires:
  ADCIq_fb/1 -> ppc/3(ADCIq_fb), Subsystem1/3(ADCIq_fb)
  Subsystem1/2(ESO) -> ESO/1
  Manual Switch/1 -> ?
  ESO+PPC/1(Iq_ref_A) -> Mux/2, Manual Switch/2
  ESO+PPC/13(g_eso_out) -> Scope/1
  ESO+PPC/14(omega_o_dyn_out) -> Scope1/1, Mux/5
  Mux/1 -> To Workspace/1
  ESO+PPC/10(iq_eso_A_out) -> Mux/3
  ESO+PPC/2(e_out) -> Mux/4
  Subsystem/1(y) -> iQ_req/1
  SpeedPU_req/1 -> Subsystem/1(SpeedPU_req), ESO+PPC/1(SpeedPU_req), Mux/1, ppc/1(SpeedPU_req), Subsystem1/1(SpeedPU_req)  "SpeedPU_req"
  SpeedPU_fdbk/1 -> ESO+PPC/2(SpeedPU_fdbk), ppc/2(SpeedPU_fdbk), Subsystem/2(SpeedPU_fdbk), Subsystem1/2(SpeedPU_fdbk)  "SpeedPU_fdbk"

== system FOCwithLOAD/Motor1 Speed control/Output Scaling ==
  DutyABC : Inport
  Data Type Conversion : DataTypeConversion  OutDataTypeStr=dataType  SaturateOnIntegerOverflow=off  RndMeth=Floor
  EnCL : DataStoreRead  DataStoreName=EnClosedLoop  IndexOptions=Index vector (dialog)  Indices=1  OutputSizes=1
  Enable : DataStoreRead  DataStoreName=AlignMode  IndexOptions=Index vector (dialog)  Indices=1  OutputSizes=1
  OrEn : Logic  Operator=OR
  PWM_Duty_Cycles : Outport
  PWM_Enable : Outport  Port=2
  wires:
  Data Type Conversion/1 -> PWM_Enable/1
  DutyABC/1 -> PWM_Duty_Cycles/1
  EnCL/1 -> OrEn/2
  OrEn/1 -> Data Type Conversion/1
  Enable/1 -> OrEn/1  "PWM_En"

== system FOCwithLOAD/Motor1 Speed control/SCI (Code Generation) ==
  SCI_Data : Inport
  Data_Conditioning_Tx : Subsystem  Variant=on
  Data_Logging : Subsystem
  Demux2 : Demux  Outputs=2
  While Iterator Subsystem : Subsystem  TreatAsAtomicUnit=on
  wires:
  Demux2/2 -> While Iterator Subsystem/2(Iteration)  "SCI_Tx_Iteration"
  Demux2/1 -> While Iterator Subsystem/1(Data)  "SCI_Tx_Data"
  SCI_Data/1 -> Data_Conditioning_Tx/1(In1)
  Data_Logging/1(SCI_Tx) -> Demux2/1
  Data_Conditioning_Tx/1(Data_Log) -> Data_Logging/1(Data_Log)

== system FOCwithLOAD/Motor1 Speed control/SCI (Simulation) ==
  SCI_Data : Inport
  Demux : Demux  Outputs=2
  Terminator1 : Terminator
  Terminator2 : Terminator
  wires:
  SCI_Data/1 -> Demux/1
  Demux/1 -> Terminator1/1
  Demux/2 -> Terminator2/1

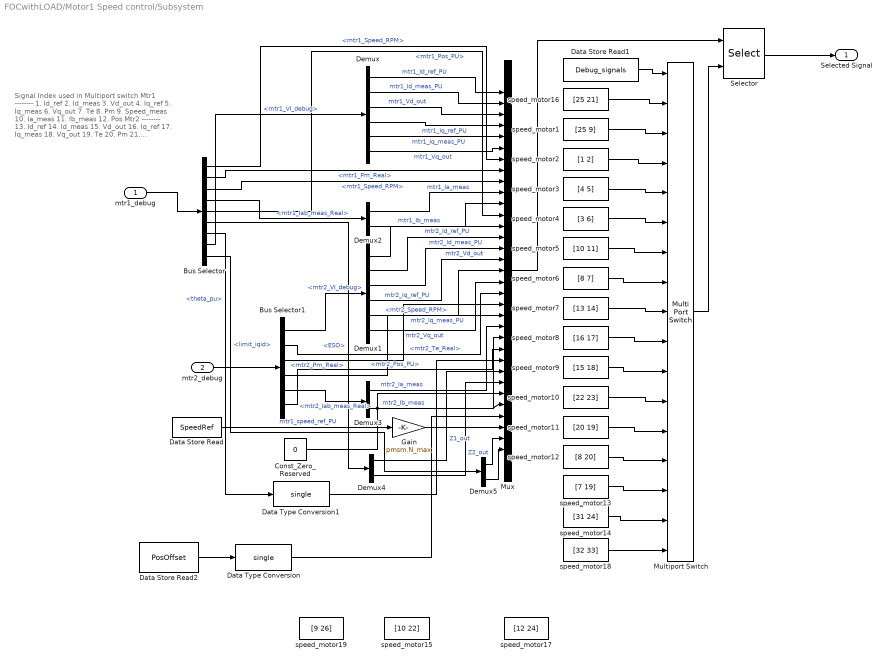
== system FOCwithLOAD/Motor1 Speed control/Subsystem ==
  note: Signal Index used in Multiport switch
      | Mtr1
      | --------
      | 1. Id_ref
      | 2. Id_meas
      | 3. Vd_out
      | 4. Iq_ref
      | 5. Iq_meas
      | 6. Vq_out
      | 7. Te
      | 8. Pm
      | 9. Speed_meas
      | 10. Ia_meas
      | 11. Ib_meas
      | 12. Pos
      |
      | Mtr2
      | --------
      | 13. Id_ref
      | 14. Id_meas
      | 15. Vd_out
      | 16. Iq_ref
      | 17. Iq_meas
      | 18. Vq_out
      | 19. Te
      | 20. Pm
      | 21. Speed_meas
      | 22. Ia_meas
      | 23. Ib_meas
      | 24. Pos
      |
      | 25.Speed ref
      |
      | 26.ESO_z1
      | 27.ESO_z2
      |
      | 28.PPC_out
  mtr1_debug : Inport
  mtr2_debug : Inport  Port=2
  Bus Selector : BusSelector  OutputSignals=mtr1_Speed_RPM,mtr1_Pm_Real,mtr1_Speed_RPM,mtr1_Iab_meas_Real,mtr1_Pos_PU,ESO,theta_pu,mtr1_VI_debug,limit_iqid
  Bus Selector1 : BusSelector  OutputSignals=mtr2_VI_debug,mtr2_Te_Real,mtr2_Pm_Real,mtr2_Speed_RPM,mtr2_Iab_meas_Real,mtr2_Pos_PU
  Const_Zero_Reserved : Constant  Value=0  OutDataTypeStr=single
  Data Store Read : DataStoreRead  DataStoreName=SpeedRef  IndexOptions=Index vector (dialog)  Indices=1  OutputSizes=1
  Data Store Read1 : DataStoreRead  DataStoreName=Debug_signals  IndexOptions=Index vector (dialog)  Indices=1  OutputSizes=1
  Data Store Read2 : DataStoreRead  DataStoreName=PosOffset  IndexOptions=Index vector (dialog)  Indices=1  OutputSizes=1
  Data Type Conversion : DataTypeConversion  OutDataTypeStr=single
  Data Type Conversion1 : DataTypeConversion  OutDataTypeStr=single  SaturateOnIntegerOverflow=off  RndMeth=Floor
  Demux : Demux  Outputs=6
  Demux1 : Demux  Outputs=6
  Demux{2..5} (4 alike) : Demux  Outputs=2
  Gain : Gain  Gain=pmsm.N_max
  Multiport Switch : MultiPortSwitch  DataPortOrder=Zero-based contiguous  Inputs=16  DiagnosticForDefault=Warning  zeroidx=on  OutDataTypeStr=uint16  RndMeth=Simplest  SaturateOnIntegerOverflow=off  InputSameDT=off
  Mux : Mux  Inputs=33
  Selector : Selector  InputPortWidth=33  IndexOptions=Index vector (port)  Indices=[1 3]  OutputSizes=1
  speed_motor1 : Constant  Value=[25 9]  OutDataTypeStr=uint16  SampleTime=-1
  speed_motor10 : Constant  Value=[22 23]  OutDataTypeStr=uint16  SampleTime=-1
  speed_motor11 : Constant  Value=[20 19]  OutDataTypeStr=uint16  SampleTime=-1
  speed_motor12 : Constant  Value=[8 20]  OutDataTypeStr=uint16  SampleTime=-1
  speed_motor13 : Constant  Value=[7 19]  OutDataTypeStr=uint16  SampleTime=-1
  speed_motor14 : Constant  Value=[31 24]  OutDataTypeStr=uint16  SampleTime=-1
  speed_motor15 : Constant  Value=[10 22]  OutDataTypeStr=uint16  SampleTime=-1
  speed_motor16 : Constant  Value=[25 21]  OutDataTypeStr=uint16  SampleTime=-1
  speed_motor17 : Constant  Value=[12 24]  OutDataTypeStr=uint16  SampleTime=-1
  speed_motor18 : Constant  Value=[32 33]  OutDataTypeStr=uint16  SampleTime=-1
  speed_motor19 : Constant  Value=[9 26]  OutDataTypeStr=uint16  SampleTime=-1
  speed_motor2 : Constant  Value=[1 2]  OutDataTypeStr=uint16  SampleTime=-1
  speed_motor3 : Constant  Value=[4 5]  OutDataTypeStr=uint16  SampleTime=-1
  speed_motor4 : Constant  Value=[3 6]  OutDataTypeStr=uint16  SampleTime=-1
  speed_motor5 : Constant  Value=[10 11]  OutDataTypeStr=uint16  SampleTime=-1
  speed_motor6 : Constant  Value=[8 7]  OutDataTypeStr=uint16  SampleTime=-1
  speed_motor7 : Constant  Value=[13 14]  OutDataTypeStr=uint16  SampleTime=-1
  speed_motor8 : Constant  Value=[16 17]  OutDataTypeStr=uint16  SampleTime=-1
  speed_motor9 : Constant  Value=[15 18]  OutDataTypeStr=uint16  SampleTime=-1
  Selected Signal : Outport
  wires:
  mtr1_debug/1 -> Bus Selector/1
  mtr2_debug/1 -> Bus Selector1/1
  Bus Selector/8 -> Demux/1  "<mtr1_VI_debug>"
  Bus Selector1/1 -> Demux1/1  "<mtr2_VI_debug>"
  Demux/1 -> Mux/1  "mtr1_Id_ref_PU"
  Demux/2 -> Mux/2  "mtr1_Id_meas_PU"
  Demux/3 -> Mux/3  "mtr1_Vd_out"
  Demux/4 -> Mux/4  "mtr1_Iq_ref_PU"
  Demux/5 -> Mux/5  "mtr1_Iq_meas_PU"
  Demux/6 -> Mux/6  "mtr1_Vq_out"
  Bus Selector/1 -> Mux/7  "<mtr1_Speed_RPM>"
  Bus Selector/2 -> Mux/8  "<mtr1_Pm_Real>"
  Bus Selector/3 -> Mux/9  "<mtr1_Speed_RPM>"
  Bus Selector/4 -> Demux2/1  "<mtr1_Iab_meas_Real>"
  Bus Selector/5 -> Mux/12  "<mtr1_Pos_PU>"
  Demux1/1 -> Mux/13  "mtr2_Id_ref_PU"
  Demux1/2 -> Mux/14  "mtr2_Id_meas_PU"
  Demux1/3 -> Mux/15  "mtr2_Vd_out"
  Demux1/4 -> Mux/16  "mtr2_Iq_ref_PU"
  Demux1/5 -> Mux/17  "mtr2_Iq_meas_PU"
  Demux1/6 -> Mux/18  "mtr2_Vq_out"
  Bus Selector1/2 -> Mux/19  "<mtr2_Te_Real>"
  Bus Selector1/3 -> Mux/20  "<mtr2_Pm_Real>"
  Bus Selector1/4 -> Mux/21  "<mtr2_Speed_RPM>"
  Bus Selector1/5 -> Demux3/1  "<mtr2_Iab_meas_Real>"
  Bus Selector1/6 -> Mux/24  "<mtr2_Pos_PU>"
  Data Store Read/1 -> Gain/1  "mtr1_speed_ref_PU"
  Mux/1 -> Selector/1
  Data Store Read1/1 -> Multiport Switch/1
  Multiport Switch/1 -> Selector/2
  Selector/1 -> Selected Signal/1
  Demux2/1 -> Mux/10  "mtr1_Ia_meas"
  Demux2/2 -> Mux/11  "mtr1_Ib_meas"
  Demux3/1 -> Mux/22  "mtr2_Ia_meas"
  Demux3/2 -> Mux/23  "mtr2_Ib_meas"
  speed_motor1/1 -> Multiport Switch/3
  speed_motor2/1 -> Multiport Switch/4
  speed_motor3/1 -> Multiport Switch/5
  speed_motor4/1 -> Multiport Switch/6
  speed_motor5/1 -> Multiport Switch/7
  speed_motor6/1 -> Multiport Switch/8
  speed_motor7/1 -> Multiport Switch/9
  speed_motor8/1 -> Multiport Switch/10
  speed_motor9/1 -> Multiport Switch/11
  speed_motor10/1 -> Multiport Switch/12
  speed_motor11/1 -> Multiport Switch/13
  speed_motor12/1 -> Multiport Switch/14
  speed_motor13/1 -> Multiport Switch/15
  speed_motor14/1 -> Multiport Switch/16
  speed_motor16/1 -> Multiport Switch/2
  Bus Selector/6 -> Demux4/1  "<ESO>"
  Gain/1 -> Mux/25
  Demux4/1 -> Mux/26  "Z1_out"
  Demux4/2 -> Mux/27  "Z2_out"
  Data Store Read2/1 -> Data Type Conversion/1
  Data Type Conversion/1 -> Mux/30
  Data Type Conversion1/1 -> Mux/31
  Bus Selector/7 -> Data Type Conversion1/1  "<theta_pu>"
  Const_Zero_Reserved/1 -> Mux/29, Mux/28
  speed_motor18/1 -> Multiport Switch/17
  Bus Selector/9 -> Demux5/1  "<limit_iqid>"
  Demux5/1 -> Mux/32
  Demux5/2 -> Mux/33

== system FOCwithLOAD/Motor1 Speed control/align ==
  real_Iq_input : Inport
  AlignReadMS : DataStoreRead  DataStoreName=AlignMode  IndexOptions=Index vector (dialog)  Indices=1  OutputSizes=1
  Data Type Conversion : DataTypeConversion  OutDataTypeStr=single  SaturateOnIntegerOverflow=off  RndMeth=Floor
  IdAlign : Constant  Value=1.5  OutDataTypeStr=single
  IdAlign1 : Constant  Value=0  OutDataTypeStr=single
  IdSw : Switch  Criteria=u2 > Threshold  Threshold=0.5  SaturateOnIntegerOverflow=off  InputSameDT=off
  IqSw : Switch  Criteria=u2 > Threshold  Threshold=0.5  SaturateOnIntegerOverflow=off  InputSameDT=off
  Mux1 : Mux  Inputs=2
  ZeroIq : Constant  Value=0  OutDataTypeStr=single
  Out1 : Outport
  wires:
  Mux1/1 -> Out1/1
  ZeroIq/1 -> IqSw/1
  IdSw/1 -> Mux1/1
  AlignReadMS/1 -> IdSw/2, IqSw/2
  IqSw/1 -> Mux1/2
  IdAlign/1 -> IdSw/1
  real_Iq_input/1 -> Data Type Conversion/1
  IdAlign1/1 -> IdSw/3
  Data Type Conversion/1 -> IqSw/3

== system FOCwithLOAD/Motor1 and Motor2 coupled/Code Generation ==
  motor1_duty : Inport
  motor2_duty : Inport  Port=2
  Gnd_m1 : Ground
  Gnd_m2 : Ground
  Term_m1 : Terminator
  Term_m2 : Terminator
  sim_fb_motor1 : Outport
  sim_fb_motor2 : Outport  Port=2
  wires:
  motor1_duty/1 -> Term_m1/1
  motor2_duty/1 -> Term_m2/1
  Gnd_m1/1 -> sim_fb_motor1/1
  Gnd_m2/1 -> sim_fb_motor2/1

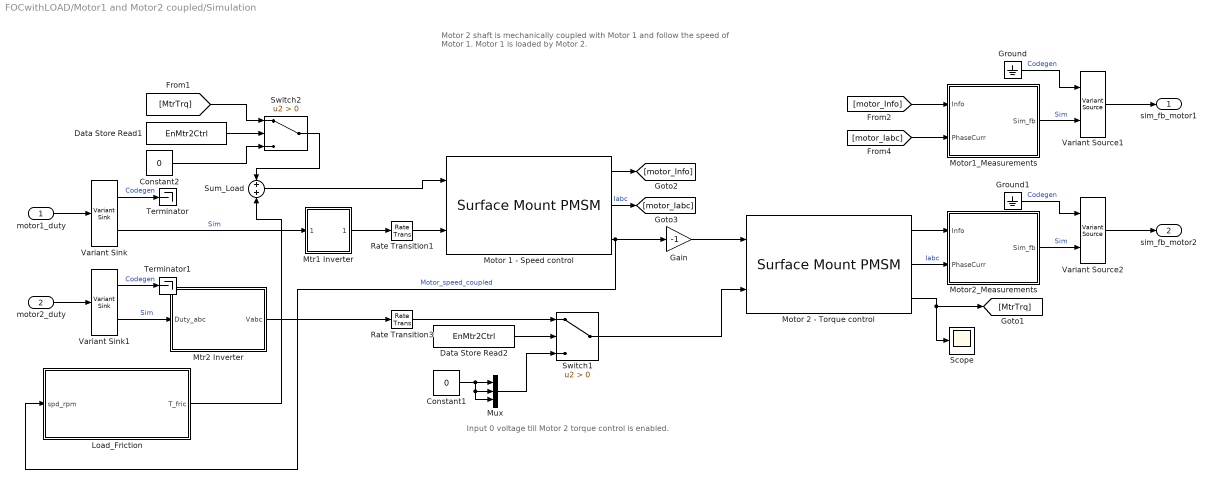
== system FOCwithLOAD/Motor1 and Motor2 coupled/Simulation ==
  note: Motor 2 shaft is mechanically coupled with Motor 1
      | and follow the speed of Motor 1.
      |
      | Motor 1 is loaded by Motor 2.
  note: Input 0 voltage till Motor 2 torque control is enabled.
  motor1_duty : Inport
  motor2_duty : Inport  Port=2
  Constant1 : Constant  Value=0
  Constant2 : Constant  Value=0
  Data Store Read1 : DataStoreRead  DataStoreName=EnMtr2Ctrl  IndexOptions=Index vector (dialog)  Indices=1  OutputSizes=1
  Data Store Read2 : DataStoreRead  DataStoreName=EnMtr2Ctrl  IndexOptions=Index vector (dialog)  Indices=1  OutputSizes=1
  Gain : Gain  Gain=-1
  Ground : Ground
  Ground1 : Ground
  Load_Friction : Subsystem
  Motor 1 - Speed control : autolibpmsmexterior/Surface Mount PMSM  port_config=Torque  sim_type=Discrete  Ts=Ts_motor  P=pmsm.p  Rs=pmsm.Rs  Ldq_=pmsm.Ld  KConstText=Permanent flux linkage constant (lambda_pm):  lambda_pm=pmsm.FluxPM  Ke=159.9771  Kt=1.323  mechanical=[pmsm.J, pmsm.B, 0]  idq0=[0 0]  theta_init=0  omega_init=0  KConst=pmsm.FluxPM  lambda_pm_calc=pmsm.FluxPM  RefBlkName='autolibpmsmexterior/Surface Mount PMSM'  aMode=5  Ldq=[pmsm.Ld pmsm.Lq]
  Motor 2 - Torque control : autolibpmsmexterior/Surface Mount PMSM  port_config=Speed  sim_type=Discrete  Ts=Ts_motor  P=pmsm2.p  Rs=pmsm2.Rs  Ldq_=pmsm2.Ld  KConstText=Permanent flux linkage constant (lambda_pm):  lambda_pm=pmsm2.FluxPM  Ke=159.9771  Kt=1.323  mechanical=[pmsm2.J, pmsm2.B, 0]  idq0=[0 0]  theta_init=0  omega_init=0  KConst=pmsm2.FluxPM  lambda_pm_calc=pmsm2.FluxPM  RefBlkName='autolibpmsmexterior/Surface Mount PMSM'  aMode=5  Ldq=[pmsm2.Ld pmsm2.Lq]
  Motor1_Measurements : Subsystem
  Motor2_Measurements : Subsystem
  Mtr1 Inverter : Subsystem
  Mtr2 Inverter : Subsystem
  Mux : Mux  Inputs=3
  Rate Transition1 : RateTransition  Deterministic=off  OutPortSampleTime=Ts_motor
  Rate Transition3 : RateTransition  Integrity=off  OutPortSampleTime=Ts_motor
  Scope : Scope
  Sum_Load : Sum
  Switch1 : Switch  Criteria=u2 > Threshold  SaturateOnIntegerOverflow=off  InputSameDT=off
  Switch2 : Switch  Criteria=u2 > Threshold  SaturateOnIntegerOverflow=off  InputSameDT=off
  Terminator : Terminator
  Terminator1 : Terminator
  Variant Sink : VariantSink  VariantControlMode=sim codegen switching
  Variant Sink1 : VariantSink  VariantControlMode=sim codegen switching
  Variant Source1 : VariantSource  VariantControlMode=sim codegen switching
  Variant Source2 : VariantSource  VariantControlMode=sim codegen switching
  sim_fb_motor1 : Outport  VectorParamsAs1DForOutWhenUnconnected=off
  sim_fb_motor2 : Outport  Port=2  VectorParamsAs1DForOutWhenUnconnected=off
  wires:
  motor1_duty/1 -> Variant Sink/1
  Variant Source1/1 -> sim_fb_motor1/1
  Motor1_Measurements/1(Sim_fb) -> Variant Source1/2  "Sim"
  Ground/1 -> Variant Source1/1  "Codegen"
  Variant Sink/1 -> Terminator/1  "Codegen"
  Rate Transition1/1 -> Motor 1 - Speed control/2
  Motor 1 - Speed control/3 -> Load_Friction/1(spd_rpm), Gain/1  "Motor_speed_coupled"
  [motor_Info] -> Motor1_Measurements/1(Info)
  [motor_Iabc] -> Motor1_Measurements/2(PhaseCurr)
  Motor 1 - Speed control/1 -> [motor_Info]
  Motor 1 - Speed control/2 -> [motor_Iabc]  "Iabc"
  Motor 2 - Torque control/1 -> Motor2_Measurements/1(Info)
  Motor 2 - Torque control/2 -> Motor2_Measurements/2(PhaseCurr)  "Iabc"
  Motor2_Measurements/1(Sim_fb) -> Variant Source2/2  "Sim"
  Mtr2 Inverter/1(Vabc) -> Rate Transition3/1
  Motor 2 - Torque control/3 -> Scope/1, [MtrTrq]
  Variant Sink1/2 -> Mtr2 Inverter/1(Duty_abc)  "Sim"
  Ground1/1 -> Variant Source2/1  "Codegen"
  Variant Source2/1 -> sim_fb_motor2/1
  motor2_duty/1 -> Variant Sink1/1
  Variant Sink1/1 -> Terminator1/1  "Codegen"
  Gain/1 -> Motor 2 - Torque control/1
  Rate Transition3/1 -> Switch1/1
  Constant2/1 -> Switch2/3
  Data Store Read1/1 -> Switch2/2
  [MtrTrq] -> Switch2/1
  Switch1/1 -> Motor 2 - Torque control/2
  Mux/1 -> Switch1/3
  Data Store Read2/1 -> Switch1/2
  Constant1/1 -> Mux/2, Mux/3, Mux/1
  Switch2/1 -> Sum_Load/1
  Load_Friction/1(T_fric) -> Sum_Load/2
  Sum_Load/1 -> Motor 1 - Speed control/1
  Mtr1 Inverter/1(Vabc) -> Rate Transition1/1
  Variant Sink/2 -> Mtr1 Inverter/1(Duty_abc)  "Sim"
